simulink model "TECMD_cycle"  (R2023a)
settings: Solver=VariableStepAuto  StartTime=0.0  StopTime=15E4  RelTol=1e-3
libraries: fl_lib x8, nesl_utility x8, BatteryLibrary_lib x2
settings Model: Creator=widana_d  LastModifiedBy=widana_d
settings DataIOCC: SaveState=on
settings DebuggingCC: UnconnectedInputMsg=warning  UnconnectedOutputMsg=warning  UnconnectedLineMsg=warning
settings ModelReferenceCC: EnableRefExpFcnMdlSchedulingChecks=on
settings RTWCC: DLArmComputeVersion=19.05

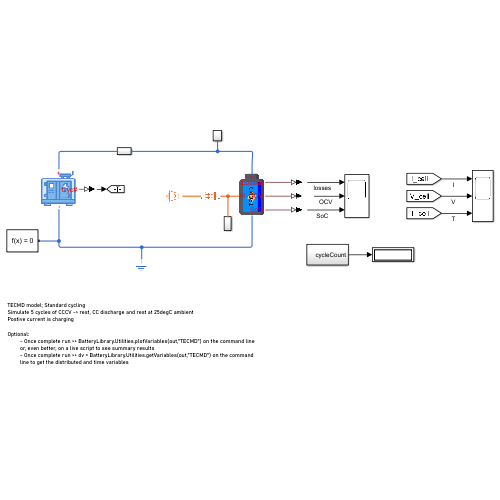
[thumbnail: Simulink's stored preview of the top-level diagram]
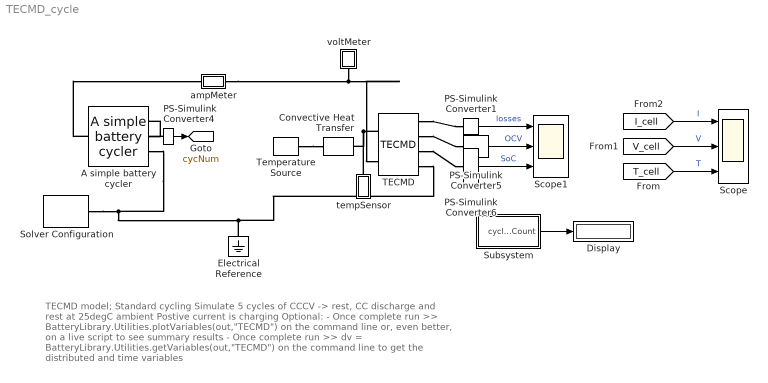
== system TECMD_cycle ==
  note: TECMD model; Standard cycling
      | Simulate 5 cycles of CCCV -> rest, CC discharge and rest at 25degC ambient
      | Postive current is charging
      |
      | Optional:
      | - Once complete run >> BatteryLibrary.Utilities.plotVariables(out,"TECMD") on the command line or, even better, on a live script to see summary results
      | - Once complete run >> dv = BatteryLibrary.Utilities.getVariables(out,"TECMD") on the command line to get the distributed and time variables
  A simple battery cycler : BatteryLibrary_lib/Utilities/A simple battery cycler  Vmax=4.2 V  Vmin=2.5 V  Ic=1.6 A  Ico=0.25 A  Id=-4.9 A  tRestC=1800 s  tRestD=3600 s
      settings: InternalSimscapePortConfiguration="{\"Bottom\":[{\"id\":\"n\",\"label\":\"-\",\"type\":\"foundation.electrical.electrical\"}],\"Left\":[],\"Right\":[{\"id\":\"numCyc\",\"label\":\"Cyc#\",\"type\":\"output\"}],\"Top\":[{\"id\":\"p\",\"label\":\"+\",\"type\":\"foundation.electrical.electrical\"}]}"
  Convective Heat Transfer : fl_lib/Thermal/Thermal Elements/Convective Heat Transfer  thermal_type=foundation.enum.constant_variable.constant  area=0.0046 m^2  heat_tr_coeff=35 W/(m^2 * K)  min_heat_tr_coeff=1e-3 W/(K*m^2)  T_specify=off  T_priority=None  T=0 K  T_nominal_specify=off  T_nominal_unit=K  T_nominal_value=1  Q_specify=off  Q_priority=None  Q=0 W  Q_nominal_specify=off  Q_nominal_unit=W  Q_nominal_value=1
  Display : Display
  Electrical Reference : fl_lib/Electrical/Electrical Elements/Electrical Reference
  PS-Simulink Converter{1,4..6} (4 alike) : nesl_utility/PS-Simulink Converter  PhysicalDomain=network_engine_domain  SubClassName=ps_output  LeftPortType=input  RightPortType=output  PseudoPeriodic=off  Frequencies=[]  VectorFormat=1-D array  Unit=inherit  AffineConversion=off
  Scope : Scope  NumInputPorts=3
  Scope1 : Scope  NumInputPorts=3
  Solver Configuration : nesl_utility/Solver Configuration  PhysicalDomain=network_engine_domain  SubClassName=solver  LeftPortType=input  RightPortType=generic  Tones=[]  Harmonics=[]  SimulateNoise=off  Profile=off  UseLocalSampling=off  EnableSwitchedLinearOptims=on  FrequencyDomain=off  UseCCode=off  RelTol=0.001  AbsTol=1e-06  MinStep=1e-09  ToWorkspace=off  RevertToSquareIcSolve=off  NumHomotopyIterations=100  PhasorMode=off  PhasorModeNumHarmonics=1  ConsistencySolver=NEWTON_FTOL  IndexReductionMethod=DerivativeReplacement  DoDC=off  ResidualTolerance=1e-09  ConsistencyTolSource=GLOBAL  ConsistencyAbsTol=0.001  ConsistencyRelTol=0.001  ConsistencyTolFactor=0.001  UseLocalSolver=off  LocalSolverChoice=NE_BACKWARD_EULER_ADVANCER  ResolveIndetEquations=on  FunctionEvalNumThread=1  LocalSolverSampleTime=0.001  DoFixedCost=off  MaxNonlinIter=3  MaxModeIter=2  ComputeImpulses=off  ImpulseIterations=2  LinearAlgebra=auto  LinearAlgebraNumThread=0  EquationFormulation=NE_TIME_EF  DelaysMemoryBudget=1024  AutomaticFiltering=on  FilteringTimeConstant=0.001  PartitionStorageMethod=AS_NEEDED  PartitionMemoryBudget=1024  PartitionMethod=ROBUST
  Subsystem : Subsystem
  TECMD : BatteryLibrary_lib/Models/TECMD  z0=0.5  T0=298 K  RoRef=12.5E-3 Ohm  RpRef=20.8E-3 Ohm  TaupRef=0.14 s  TauRef=580 s  Cn=4.9 hr*A  Cp=110 J/K  Tref=298 K  Ea_Ro=8.013 kJ/mol  Ea_Rp=9.12 kJ/mol  Ea_Taup=9.79 kJ/mol  Ea_Tau=27 kJ/mol  refSoC=[0 : 100]' / 100  refOCV=[2.87226666666667, 2.96052812994699, 3.02804006137187, 3.09555199279676, 3.16306392422164, 3.2001291114499, 3.22684932876092, 3.25356954607195, 3.28028976338298, 3.30366251902926, 3.32391086783852, 3.34415921664777, 3.36440756545703, 3.38337736980428, 3.39585056120364, 3.40808169748128, 3.42031283375891, 3.43312236542483, 3.44403277212358, 3.45436831838031, 3.46470386463704, 3.47489460441589, 3.48578295282009, 3.49716895836194, 3.50855496390379, 3.51975057723135, 3.52990789728309, 3.54012269726924, 3.55033749725539, 3.56053403978798, 3.56876876393151, 3.57634734074831, 3.58392591756512, 3.59150449438192, 3.59837651292555, 3.60400711532064, 3.60963771771574, 3.61526832011083, 3.62087603938814, 3.62605990154572, 3.63124376370329, 3.63642762586086, 3.64172472997681, 3.64738310137943, 3.65304989960037, 3.6587166978213, 3.66472767182913, 3.67174598798367, 3.6788777371365, 3.68600948628932, 3.69349161904363, 3.7024953271603, 3.7118125338251, 3.7211297404899, 3.73077493215115, 3.74281715264455, 3.75539849306634, 3.76797983348813, 3.78054451462135, 3.79302677795269, 3.80637677297635, 3.81972676800001, 3.83307676302367, 3.84456984787373, 3.85430164068239, 3.86403343349106, 3.87376522629972, 3.88293282901064, 3.89107889951479, 3.89922497001894, 3.90737104052308, 3.91557874276785, 3.92399213081386, 3.93240787383325, 3.94082361685263, 3.94963150612215, 3.95966546646635, 3.96983594392408, 3.98000642138181, 3.99032598576655, 4.00126821478467, 4.01233626061718, 4.02340430644969, 4.03432201816434, 4.04382704177779, 4.05280216094291, 4.06177728010803, 4.07065703360974, 4.07626015949775, 4.08051431663774, 4.08476847377773, 4.08902263091772, 4.09345555380871, 4.09831742254355, 4.1031792912784, 4.10804116001324, 4.1155790937363, 4.12906316200268, 4.14254723026907, 4.15856111602972, 4.17532536875376]' V
      settings: InternalSimscapePortConfiguration="{\"Bottom\":[{\"id\":\"n\",\"label\":\"-\",\"type\":\"foundation.electrical.electrical\"}],\"Left\":[{\"id\":\"Hi\",\"label\":\"H\",\"type\":\"foundation.thermal.thermal\"}],\"Right\":[{\"id\":\"eta\",\"label\":\"Losses\",\"type\":\"output\"},{\"id\":\"OCV\",\"label\":\"OCV\",\"type\":\"output\"},{\"id\":\"zbar\",\"label\":\"SoC\",\"type\":\"output\"}],\"Top\":[{\"id\":\"p\",\"label\":\"+\",\"type\":\"foundation.electrical.electrical\"}]}"
  Temperature Source : fl_lib/Thermal/Thermal Sources/Temperature Source  temperature=25 degC
  ampMeter : Subsystem
  tempSensor : Subsystem
  voltMeter : Subsystem
  tag scope: cycNum=global
  wires:
  PS-Simulink Converter4/1 -> [cycNum]
  Subsystem/1(cycleCount) -> Display/1
  PS-Simulink Converter6/1 -> Scope1/3  "SoC"
  PS-Simulink Converter1/1 -> Scope1/1  "losses"
  PS-Simulink Converter5/1 -> Scope1/2  "OCV"
  [V_cell] -> Scope/2  "V"
  [I_cell] -> Scope/1  "I"
  [T_cell] -> Scope/3  "T"
  connections:
  ampMeter/RConn1 -- TECMD/LConn2 -- voltMeter/LConn1
  Electrical Reference/LConn1 -- Solver Configuration/RConn1 -- A simple battery cycler/RConn2 -- TECMD/RConn4
  TECMD/LConn1 -- Convective Heat Transfer/LConn1 -- tempSensor/LConn1
  Temperature Source/LConn1 -- Convective Heat Transfer/RConn1
  PS-Simulink Converter4/LConn1 -- A simple battery cycler/RConn1
  A simple battery cycler/LConn1 -- ampMeter/LConn1
  TECMD/RConn3 -- PS-Simulink Converter6/LConn1
  TECMD/RConn2 -- PS-Simulink Converter5/LConn1
  TECMD/RConn1 -- PS-Simulink Converter1/LConn1

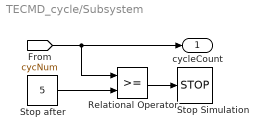
== system TECMD_cycle/Subsystem ==
  Relational Operator : RelationalOperator  OutDataTypeStr=boolean  RndMeth=Simplest  InputSameDT=off
  Stop Simulation : Stop
  Stop after : Constant  Value=5
  cycleCount : Outport
  wires:
  Stop after/1 -> Relational Operator/2
  [cycNum] -> Relational Operator/1, cycleCount/1
  Relational Operator/1 -> Stop Simulation/1

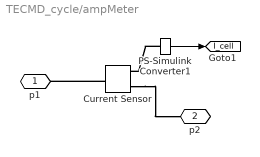
== system TECMD_cycle/ampMeter ==
  Current Sensor : fl_lib/Electrical/Electrical Sensors/Current Sensor
  PS-Simulink Converter1 : nesl_utility/PS-Simulink Converter  PhysicalDomain=network_engine_domain  SubClassName=ps_output  LeftPortType=input  RightPortType=output  PseudoPeriodic=off  Frequencies=[]  VectorFormat=1-D array  Unit=inherit  AffineConversion=off
  p1 : PMIOPort  Side=Left
  p2 : PMIOPort  Port=2  Side=Right
  tag scope: I_cell=global
  wires:
  PS-Simulink Converter1/1 -> [I_cell]
  connections:
  Current Sensor/RConn2 -- p2/RConn1
  Current Sensor/LConn1 -- p1/RConn1
  PS-Simulink Converter1/LConn1 -- Current Sensor/RConn1

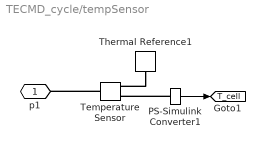
== system TECMD_cycle/tempSensor ==
  PS-Simulink Converter1 : nesl_utility/PS-Simulink Converter  PhysicalDomain=network_engine_domain  SubClassName=ps_output  LeftPortType=input  RightPortType=output  PseudoPeriodic=off  Frequencies=[]  VectorFormat=1-D array  Unit=inherit  AffineConversion=off
  Temperature Sensor : fl_lib/Thermal/Thermal Sensors/Temperature Sensor  temperature_measure=foundation.enum.MeasurementReference.difference
  Thermal Reference1 : fl_lib/Thermal/Thermal Elements/Thermal Reference
  p1 : PMIOPort  Side=Left
  tag scope: T_cell=global
  wires:
  PS-Simulink Converter1/1 -> [T_cell]
  connections:
  Temperature Sensor/LConn1 -- p1/RConn1
  PS-Simulink Converter1/LConn1 -- Temperature Sensor/RConn2
  Thermal Reference1/LConn1 -- Temperature Sensor/RConn1

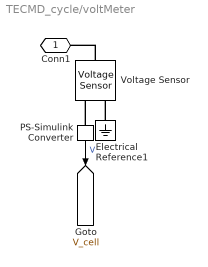
== system TECMD_cycle/voltMeter ==
  Electrical Reference1 : fl_lib/Electrical/Electrical Elements/Electrical Reference
  PS-Simulink Converter : nesl_utility/PS-Simulink Converter  PhysicalDomain=network_engine_domain  SubClassName=ps_output  LeftPortType=input  RightPortType=output  PseudoPeriodic=off  Frequencies=[]  VectorFormat=1-D array  Unit=inherit  AffineConversion=off
  Voltage Sensor : fl_lib/Electrical/Electrical Sensors/Voltage Sensor
  Conn1 : PMIOPort  Side=Left
  tag scope: V_cell=global
  wires:
  PS-Simulink Converter/1 -> [V_cell]  "V"
  connections:
  Voltage Sensor/LConn1 -- Conn1/RConn1
  PS-Simulink Converter/LConn1 -- Voltage Sensor/RConn1
  Electrical Reference1/LConn1 -- Voltage Sensor/RConn2
